simulink model "QuadCopter"  (R2022b)
settings: Solver=ode45  StartTime=0.0  StopTime=500  MaxStep=0.01  RelTol=1e-3
StopFcn:
  | plot3dir(out.X_LQR.x1_or_X__LQR_,out.X_LQR.x2_or_Y, out.X_LQR.x3_or_Z);
  | plot3dir(out.X_MPC.x1_or_X_MPC_,out.X_MPC.x2_or_Y,out.X_MPC.x3_or_Z)
values from neighbouring files (symbols this model uses):
  Fmpc = [0 0 0.003136 0 0 0 0.0020575296 0 0 0 0.0012845056 0 ... (480 elements, 40x12)]    [Fmpc.mat]    (also in FmpcNew.mat = [-6.41677792694e-13 -2.592942847e-12 12.5317858023 -7.722638; dataMPC.m = 2*SuN'*Qbar*Sx)
  g = 9.8    [A.mat]    (also in dataLQR.m)
  Hmpc = [2.0029864 0 0 0 0.00268248 0 0 0 0.00237888 0 0 0 ... (1600 elements, 40x40)]    [Hmpc.mat]    (also in HmpcNew.mat = [2.75081323273 -2.14300187551e-15 -2.22961409187e-14 -3.9742; dataMPC.m = (Hmpc + Hmpc')/2)
  Ix = 0.005    [A.mat]    (also in dataLQR.m)
  Iy = 0.005    [A.mat]    (also in dataLQR.m)
  Iz = 0.009    [A.mat]    (also in dataLQR.m)
  K = [1.7040962205e-15 -3.44587222128e-18 0.005 -1.12753414634e-18 -5.98079995663e-16 -0.005 -2.65215557868e-18 5.41102545065e-19 2 -9.36752747927e-18 -1.48674599099e-17 1.40946704004e-18 ... (48 elements, 4x12)]    [K.mat]
  kf = 1e-05    [A.mat]    (also in dataLQR.m)
  km = 1e-07    [A.mat]    (also in dataLQR.m)
  l = 0.2    [A.mat]    (also in dataLQR.m)
  M = 0.5    [A.mat]    (also in dataLQR.m)
libraries: PID_costum x4
CloseFcn:
  | plot3dir(out.X_LQR.x1_or_X__LQR_,out.X_LQR.x2_or_Y, out.X_LQR.x3_or_Z);
  | plot3dir(out.X_MPC.x1_or_X_MPC_,out.X_MPC.x2_or_Y,out.X_MPC.x3_or_Z)
settings Model: Creator=asoltanieh  LastModifiedBy=asoltanieh

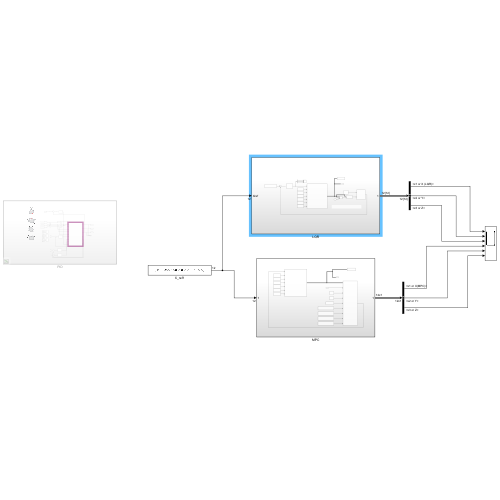
[thumbnail: Simulink's stored preview of the top-level diagram]
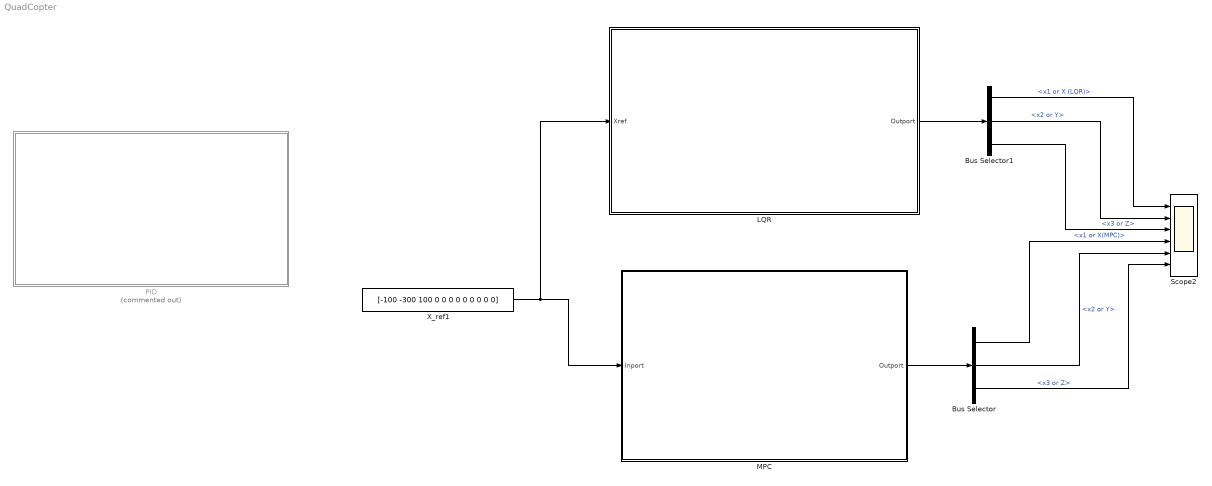
== system QuadCopter ==
  Bus Selector : BusSelector  OutputSignals=x1 or X(MPC),x2 or Y,x3 or Z
  Bus Selector1 : BusSelector  OutputSignals=x1 or X (LQR),x2 or Y,x3 or Z
  LQR : Subsystem
  MPC : Subsystem
  PID : Subsystem  Commented=on
  Scope2 : Scope  NumInputPorts=6
  X_ref1 : Constant  Value=[-100 -300 100 0 0 0 0 0 0 0 0 0]
  wires:
  Bus Selector/2 -> Scope2/5  "<x2 or Y>"
  Bus Selector/1 -> Scope2/4  "<x1 or X(MPC)>"
  Bus Selector/3 -> Scope2/6  "<x3 or Z>"
  MPC/1(Outport) -> Bus Selector/1
  LQR/1(Outport) -> Bus Selector1/1
  Bus Selector1/3 -> Scope2/3  "<x3 or Z>"
  Bus Selector1/1 -> Scope2/1  "<x1 or X (LQR)>"
  Bus Selector1/2 -> Scope2/2  "<x2 or Y>"
  X_ref1/1 -> LQR/1(Xref), MPC/1(Inport)

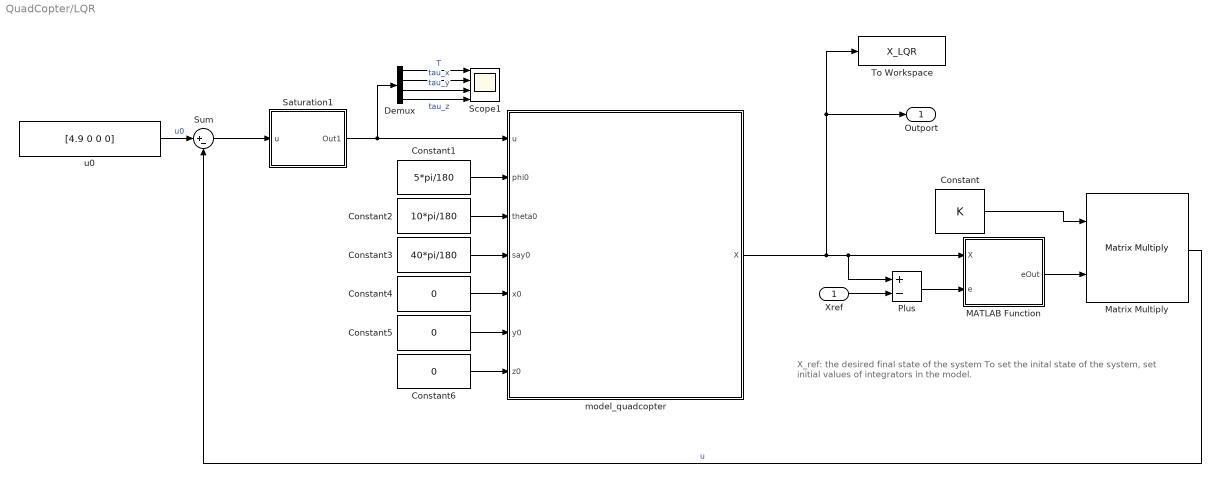
== system QuadCopter/LQR ==
  note: X_ref: the desired final state of the system
      |
      | To set the inital state of the system, set initial values of integrators in the model.
  Xref : Inport
  Constant : Constant  Value=K
  Constant1 : Constant  Value=5*pi/180
  Constant2 : Constant  Value=10*pi/180
  Constant3 : Constant  Value=40*pi/180
  Constant4 : Constant  Value=0
  Constant5 : Constant  Value=0
  Constant6 : Constant  Value=0
  Demux : Demux
  MATLAB Function : MATLAB Function  TreatAsAtomicUnit=on
  Matrix Multiply : Product  Multiplication=Matrix(*)
  Plus : Sum  Inputs=+-
  Saturation1 : Subsystem
  Scope1 : Scope  NumInputPorts=4
  Sum : Sum  Inputs=|+-
  To Workspace : ToWorkspace  VariableName=X_LQR  SaveFormat=Timeseries  SampleTime=-1
  model_quadcopter : Subsystem
  u0 : Constant  Value=[4.9 0 0 0]
  Outport : Outport
  wires:
  model_quadcopter/1(X) -> MATLAB Function/1(X), Plus/1, Outport/1, To Workspace/1
  Constant/1 -> Matrix Multiply/1
  u0/1 -> Sum/1  "u0"
  Sum/1 -> Saturation1/1(u)
  Plus/1 -> MATLAB Function/2(e)
  Xref/1 -> Plus/2
  Demux/1 -> Scope1/1  "T"
  Demux/2 -> Scope1/2  "tau_x"
  Demux/3 -> Scope1/3  "tau_y"
  Demux/4 -> Scope1/4  "tau_z"
  Matrix Multiply/1 -> Sum/2  "u"
  Constant1/1 -> model_quadcopter/2(phi0)
  Constant3/1 -> model_quadcopter/4(say0)
  Constant2/1 -> model_quadcopter/3(theta0)
  Constant4/1 -> model_quadcopter/5(x0)
  Constant5/1 -> model_quadcopter/6(y0)
  Constant6/1 -> model_quadcopter/7(z0)
  Saturation1/1(Out1) -> Demux/1, model_quadcopter/1(u)
  MATLAB Function/1(eOut) -> Matrix Multiply/2

== system QuadCopter/MPC ==
  Inport : Inport
  Constant : Constant  Value=Hmpc
  Constant1 : Constant  Value=Fmpc
  Constant2 : Constant  Value=0.088946471
  Constant3 : Constant  Value=5*pi/180
  Constant4 : Constant  Value=10*pi/180
  Constant5 : Constant  Value=40*pi/180
  Constant6 : Constant  Value=0
  Constant7 : Constant  Value=0
  Constant8 : Constant  Value=0
  MATLAB Function : MATLAB Function  TreatAsAtomicUnit=on
  To Workspace : ToWorkspace  VariableName=X_MPC  SaveFormat=Timeseries  SampleTime=-1
  model_quadcopter : Subsystem
  u0 : Constant  Value=[4.9 0 0 0]
  umax : Constant  Value=[10; 0.01; 0.01; 0.002]
  umin : Constant  Value=[0; -0.01; -0.01; -0.002]
  uscale : Constant  Value=[0.5; 0.003; 0.003; 0.0006]
  Outport : Outport
  wires:
  MATLAB Function/1(U) -> model_quadcopter/1(u)
  Inport/1 -> MATLAB Function/2(Xref)
  Constant/1 -> MATLAB Function/3(Hmpc)
  Constant1/1 -> MATLAB Function/4(Fmpc)
  u0/1 -> MATLAB Function/6(U0)
  Constant2/1 -> MATLAB Function/5(alpha)
  umin/1 -> MATLAB Function/7(Umin)
  umax/1 -> MATLAB Function/8(Umax)
  uscale/1 -> MATLAB Function/9(uScale)
  model_quadcopter/1(X) -> MATLAB Function/1(X), Outport/1, To Workspace/1
  Constant4/1 -> model_quadcopter/3(theta0)
  Constant3/1 -> model_quadcopter/2(phi0)
  Constant8/1 -> model_quadcopter/7(z0)
  Constant7/1 -> model_quadcopter/6(y0)
  Constant5/1 -> model_quadcopter/4(say0)
  Constant6/1 -> model_quadcopter/5(x0)

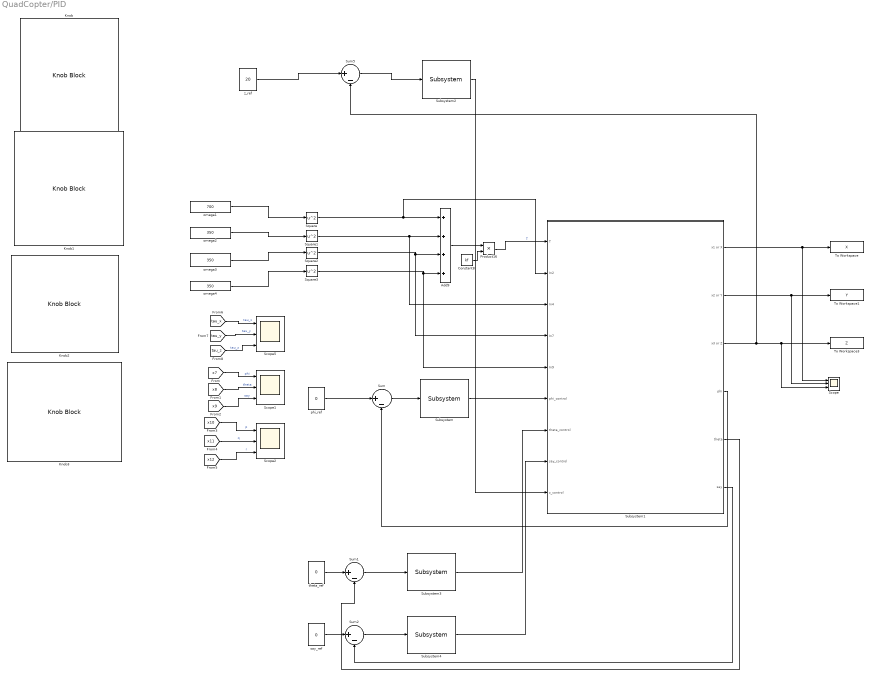
== system QuadCopter/PID ==
  Add9 : Sum  Inputs=++++
  Constant8 : Constant  Value=kf
  Knob{,1..3} (4 alike) : KnobBlock  ScaleMax=700
  Product16 : Product
  Scope{,1..2,5} (4 alike) : Scope  NumInputPorts=3
  Square{,1..3} (4 alike) : Math  Operator=square
  Subsystem : PID_costum/Subsystem  K_P=0.08  K_I=0  K_D=0.032  Sat_value=0.5
  Subsystem1 : Subsystem
  Subsystem2 : PID_costum/Subsystem  K_P=5  K_I=1  K_D=2  Sat_value=10
  Subsystem3 : PID_costum/Subsystem  K_P=0.08  K_I=0  K_D=0.032  Sat_value=0.5
  Subsystem4 : PID_costum/Subsystem  K_P=0.04  K_I=0  K_D=0.07  Sat_value=0.1
  Sum{,1..2,5} (4 alike) : Sum  Inputs=|+-
  To Workspace : ToWorkspace  VariableName=X  SampleTime=-1
  To Workspace1 : ToWorkspace  VariableName=Y  SampleTime=-1
  To Workspace3 : ToWorkspace  VariableName=Z  SampleTime=-1
  omega1 : Constant  Value=700
  omega2 : Constant  Value=350
  omega3 : Constant  Value=350
  omega4 : Constant  Value=350
  phi_ref : Constant  Value=0
  say_ref : Constant  Value=0
  theta_ref : Constant  Value=0
  z_ref : Constant  Value=20
  wires:
  Subsystem1/2(x2 or Y) -> Scope/2, To Workspace1/1
  Product16/1 -> Subsystem1/1(T)  "T"
  [x12] -> Scope2/3  "r"
  [x10] -> Scope2/1  "p"
  Square3/1 -> Subsystem1/5(In9), Add9/4
  [tau_x] -> Scope5/1  "tau_x"
  Subsystem1/4(phi) -> Sum/2
  Subsystem1/3(x3 or Z) -> Sum5/2, Scope/3, To Workspace3/1
  [x11] -> Scope2/2  "q"
  [tau_z] -> Scope5/3  "tau_z"
  [tau_y] -> Scope5/2  "tau_y"
  Square2/1 -> Subsystem1/4(In7), Add9/3
  [x7] -> Scope1/1  "phi"
  Square/1 -> Subsystem1/2(In2), Add9/1
  Subsystem1/6(say) -> Sum2/2
  z_ref/1 -> Sum5/1
  [x9] -> Scope1/3  "say"
  omega1/1 -> Square/1
  Add9/1 -> Product16/1
  Square1/1 -> Subsystem1/3(In4), Add9/2
  Constant8/1 -> Product16/2
  phi_ref/1 -> Sum/1
  say_ref/1 -> Sum2/1
  Subsystem1/1(x1 or X) -> Scope/1, To Workspace/1
  Subsystem/1 -> Subsystem1/6(phi_control)
  Sum/1 -> Subsystem/1
  omega4/1 -> Square3/1
  omega3/1 -> Square2/1
  Sum1/1 -> Subsystem3/1
  Sum5/1 -> Subsystem2/1
  Subsystem3/1 -> Subsystem1/7(theta_control)
  omega2/1 -> Square1/1
  Subsystem1/5(theta) -> Sum1/2
  Subsystem4/1 -> Subsystem1/8(say_control)
  theta_ref/1 -> Sum1/1
  Subsystem2/1 -> Subsystem1/9(z_control)
  [x8] -> Scope1/2  "theta"
  Sum2/1 -> Subsystem4/1

== system QuadCopter/LQR/Saturation1 ==
  u : Inport
  Demux1 : Demux
  Saturation : Saturate  UpperLimit=10  LowerLimit=0
  Saturation1 : Saturate  UpperLimit=0.01  LowerLimit=-0.01
  Saturation2 : Saturate  UpperLimit=0.01  LowerLimit=-0.01
  Saturation3 : Saturate  UpperLimit=0.002  LowerLimit=-0.002
  Vector Concatenate : Concatenate  NumInputs=4
  Out1 : Outport
  wires:
  Vector Concatenate/1 -> Out1/1
  u/1 -> Demux1/1
  Saturation2/1 -> Vector Concatenate/3
  Saturation/1 -> Vector Concatenate/1
  Demux1/1 -> Saturation/1
  Demux1/4 -> Saturation3/1
  Demux1/2 -> Saturation1/1
  Saturation1/1 -> Vector Concatenate/2
  Saturation3/1 -> Vector Concatenate/4
  Demux1/3 -> Saturation2/1

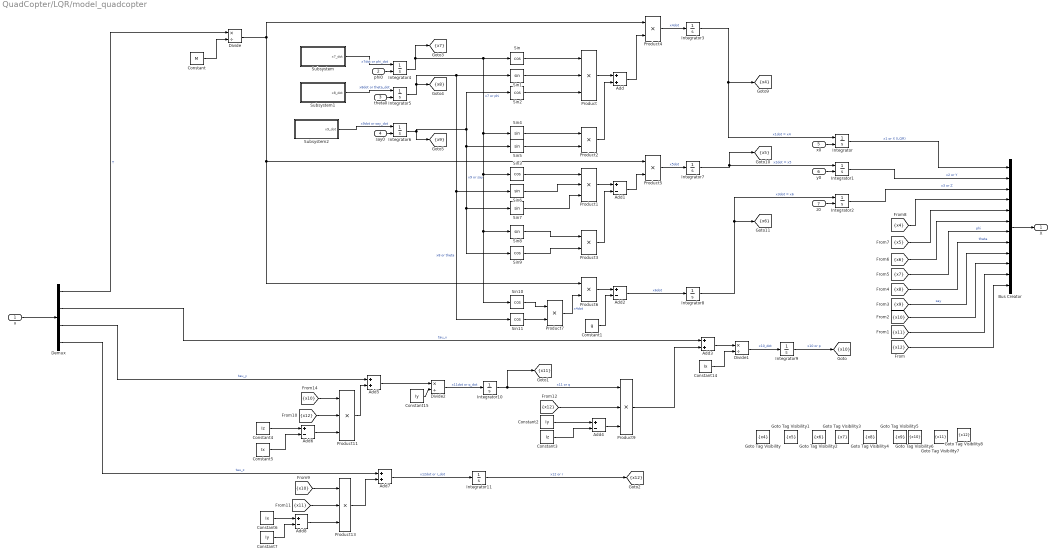
== system QuadCopter/LQR/model_quadcopter ==
  u : Inport
  phi0 : Inport  Port=2
  theta0 : Inport  Port=3
  say0 : Inport  Port=4
  x0 : Inport  Port=5
  y0 : Inport  Port=6
  z0 : Inport  Port=7
  Add{,3,5,7} (4 alike) : Sum
  Add{1..2,4,6,8} (5 alike) : Sum  Inputs=+-
  Bus Creator : BusCreator  Inputs=12
  Constant : Constant  Value=M
  Constant1 : Constant  Value=g
  Constant14 : Constant  Value=Ix
  Constant15 : Constant  Value=Iy
  Constant2 : Constant  Value=Iy
  Constant3 : Constant  Value=Iz
  Constant4 : Constant  Value=Iz
  Constant5 : Constant  Value=Ix
  Constant6 : Constant  Value=Ix
  Constant7 : Constant  Value=Iy
  Demux : Demux
  Divide : Product  Inputs=*/
  Divide1 : Product  Inputs=*/
  Divide2 : Product  Inputs=*/
  Goto Tag Visibility : GotoTagVisibility  GotoTag=x4
  Goto Tag Visibility1 : GotoTagVisibility  GotoTag=x5
  Goto Tag Visibility2 : GotoTagVisibility  GotoTag=x6
  Goto Tag Visibility3 : GotoTagVisibility  GotoTag=x7
  Goto Tag Visibility4 : GotoTagVisibility  GotoTag=x8
  Goto Tag Visibility5 : GotoTagVisibility  GotoTag=x9
  Goto Tag Visibility6 : GotoTagVisibility  GotoTag=x10
  Goto Tag Visibility7 : GotoTagVisibility  GotoTag=x11
  Goto Tag Visibility8 : GotoTagVisibility  GotoTag=x12
  Integrator : Integrator  InitialConditionSource=external  InitialCondition=2
  Integrator1 : Integrator  InitialConditionSource=external  InitialCondition=5
  Integrator{3,7..11} (6 alike) : Integrator
  Integrator2 : Integrator  InitialConditionSource=external  InitialCondition=-1
  Integrator4 : Integrator  InitialConditionSource=external  InitialCondition=20*pi/180
  Integrator5 : Integrator  InitialConditionSource=external  InitialCondition=30*pi/180
  Integrator6 : Integrator  InitialConditionSource=external  InitialCondition=45*pi/180
  Product{,1,9,11,13} (5 alike) : Product  Inputs=3
  Product{2..7} (6 alike) : Product
  Sin{,2..3,9..11} (6 alike) : Trigonometry  Operator=cos
  Sin{1,4..8} (6 alike) : Trigonometry
  Subsystem : Subsystem
  Subsystem1 : Subsystem
  Subsystem2 : Subsystem
  X : Outport
  tag scope: x10=scoped, x11=scoped, x12=scoped, x4=scoped, x5=scoped, x6=scoped, x7=scoped, x8=scoped, x9=scoped
  wires:
  Constant7/1 -> Add8/2
  Product/1 -> Add/1
  Integrator7/1 -> [x5], Integrator1/1  "x2dot = x5"
  Demux/2 -> Add3/1  "tau_x"
  Product7/1 -> Product6/2  "x4dot"
  Add6/1 -> Product11/3
  Add8/1 -> Product13/3
  Demux/4 -> Add7/1  "tau_z"
  Constant14/1 -> Divide1/2
  Divide/1 -> Product6/1, Product5/1, Product4/1
  Integrator6/1 -> Sin2/1, Sin9/1, Sin7/1, Sin5/1, [x9]  "x9 or say"
  Constant3/1 -> Add4/2
  [x10] -> Product13/1
  Divide2/1 -> Integrator10/1  "x11dot or q_dot"
  Add4/1 -> Product9/3
  Subsystem1/1(x8_dot) -> Integrator5/1  "x8dot or theta_dot"
  Product13/1 -> Add7/2
  Constant/1 -> Divide/2
  Integrator10/1 -> [x11], Product9/1  "x11 or q"
  [x11] -> Product13/2
  Sin2/1 -> Product/3
  Constant6/1 -> Add8/1
  Sin/1 -> Product/1
  Sin11/1 -> Product7/2
  Sin6/1 -> Product1/2
  Subsystem/1(x7_dot) -> Integrator4/1  "x7dot or phi_dot"
  Product11/1 -> Add5/2
  Constant2/1 -> Add4/1
  Sin1/1 -> Product/2
  Integrator5/1 -> Sin11/1, Sin6/1, Sin1/1, [x8]  "x8 or theta"
  Sin10/1 -> Product7/1
  Add5/1 -> Divide2/1
  Product3/1 -> Add1/2
  Subsystem2/1(x9_dot) -> Integrator6/1  "x9dot or say_dot"
  Add7/1 -> Integrator11/1  "x12dot or r_dot"
  Add2/1 -> Integrator8/1  "x6dot"
  Add1/1 -> Product5/2
  Constant4/1 -> Add6/1
  Sin3/1 -> Product1/1
  Divide1/1 -> Integrator9/1  "x10_dot"
  [x12] -> Product9/2
  Sin7/1 -> Product1/3
  Product5/1 -> Integrator7/1  "x5dot"
  [x12] -> Product11/2
  Constant15/1 -> Divide2/2
  Product9/1 -> Add3/2
  Integrator4/1 -> Sin10/1, Sin8/1, Sin3/1, Sin4/1, Sin/1, [x7]  "x7 or phi"
  Add3/1 -> Divide1/1
  Integrator3/1 -> [x4], Integrator/1  "x1dot = x4"
  Sin8/1 -> Product3/1
  Sin4/1 -> Product2/1
  Product6/1 -> Add2/1
  [x10] -> Product11/1
  Integrator9/1 -> [x10]  "x10 or p"
  Product1/1 -> Add1/1
  Integrator8/1 -> [x6], Integrator2/1  "x3dot = x6"
  Sin5/1 -> Product2/2
  Constant1/1 -> Add2/2
  Demux/3 -> Add5/1  "tau_y"
  Constant5/1 -> Add6/2
  Add/1 -> Product4/2
  Product2/1 -> Add/2
  Sin9/1 -> Product3/2
  Product4/1 -> Integrator3/1  "x4dot"
  Integrator11/1 -> [x12]  "x12 or r"
  Demux/1 -> Divide/1  "T"
  Bus Creator/1 -> X/1
  u/1 -> Demux/1
  Integrator1/1 -> Bus Creator/2  "x2 or Y"
  Integrator2/1 -> Bus Creator/3  "x3 or Z"
  Integrator/1 -> Bus Creator/1  "x1 or X (LQR)"
  [x4] -> Bus Creator/4
  [x5] -> Bus Creator/5
  [x6] -> Bus Creator/6
  [x7] -> Bus Creator/7  "phi"
  [x8] -> Bus Creator/8  "theta"
  [x9] -> Bus Creator/9  "say"
  [x10] -> Bus Creator/10
  [x11] -> Bus Creator/11
  [x12] -> Bus Creator/12
  phi0/1 -> Integrator4/2
  theta0/1 -> Integrator5/2
  say0/1 -> Integrator6/2
  x0/1 -> Integrator/2
  y0/1 -> Integrator1/2
  z0/1 -> Integrator2/2

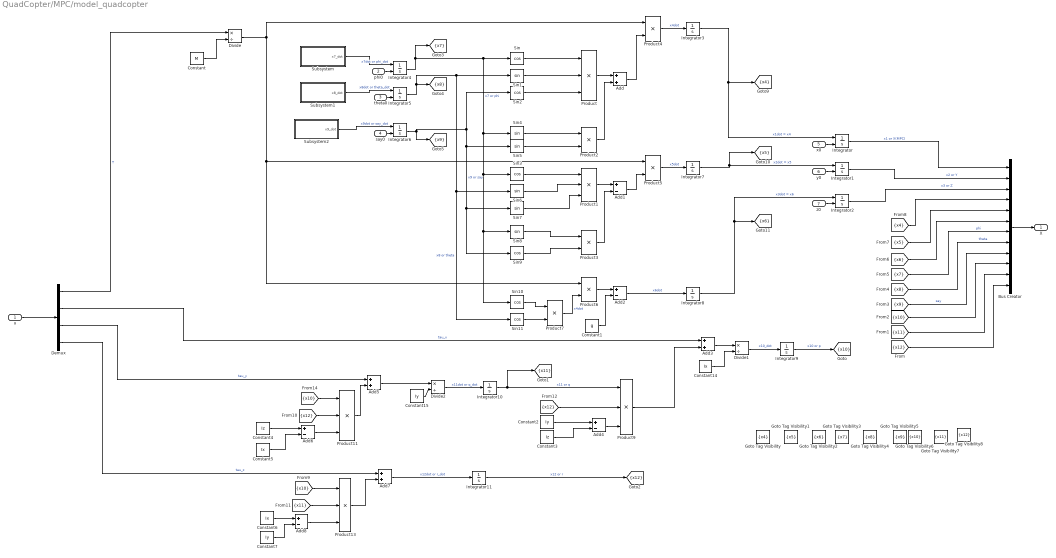
== system QuadCopter/MPC/model_quadcopter ==
  u : Inport
  phi0 : Inport  Port=2
  theta0 : Inport  Port=3
  say0 : Inport  Port=4
  x0 : Inport  Port=5
  y0 : Inport  Port=6
  z0 : Inport  Port=7
  Add{,3,5,7} (4 alike) : Sum
  Add{1..2,4,6,8} (5 alike) : Sum  Inputs=+-
  Bus Creator : BusCreator  Inputs=12
  Constant : Constant  Value=M
  Constant1 : Constant  Value=g
  Constant14 : Constant  Value=Ix
  Constant15 : Constant  Value=Iy
  Constant2 : Constant  Value=Iy
  Constant3 : Constant  Value=Iz
  Constant4 : Constant  Value=Iz
  Constant5 : Constant  Value=Ix
  Constant6 : Constant  Value=Ix
  Constant7 : Constant  Value=Iy
  Demux : Demux
  Divide : Product  Inputs=*/
  Divide1 : Product  Inputs=*/
  Divide2 : Product  Inputs=*/
  Goto Tag Visibility : GotoTagVisibility  GotoTag=x4
  Goto Tag Visibility1 : GotoTagVisibility  GotoTag=x5
  Goto Tag Visibility2 : GotoTagVisibility  GotoTag=x6
  Goto Tag Visibility3 : GotoTagVisibility  GotoTag=x7
  Goto Tag Visibility4 : GotoTagVisibility  GotoTag=x8
  Goto Tag Visibility5 : GotoTagVisibility  GotoTag=x9
  Goto Tag Visibility6 : GotoTagVisibility  GotoTag=x10
  Goto Tag Visibility7 : GotoTagVisibility  GotoTag=x11
  Goto Tag Visibility8 : GotoTagVisibility  GotoTag=x12
  Integrator : Integrator  InitialConditionSource=external  InitialCondition=2
  Integrator1 : Integrator  InitialConditionSource=external  InitialCondition=5
  Integrator{3,7..11} (6 alike) : Integrator
  Integrator2 : Integrator  InitialConditionSource=external  InitialCondition=-1
  Integrator4 : Integrator  InitialConditionSource=external  InitialCondition=20*pi/180
  Integrator5 : Integrator  InitialConditionSource=external  InitialCondition=30*pi/180
  Integrator6 : Integrator  InitialConditionSource=external  InitialCondition=45*pi/180
  Product{,1,9,11,13} (5 alike) : Product  Inputs=3
  Product{2..7} (6 alike) : Product
  Sin{,2..3,9..11} (6 alike) : Trigonometry  Operator=cos
  Sin{1,4..8} (6 alike) : Trigonometry
  Subsystem : Subsystem
  Subsystem1 : Subsystem
  Subsystem2 : Subsystem
  X : Outport
  tag scope: x10=scoped, x11=scoped, x12=scoped, x4=scoped, x5=scoped, x6=scoped, x7=scoped, x8=scoped, x9=scoped
  wires:
  Constant7/1 -> Add8/2
  Product/1 -> Add/1
  Integrator7/1 -> [x5], Integrator1/1  "x2dot = x5"
  Demux/2 -> Add3/1  "tau_x"
  Product7/1 -> Product6/2  "x4dot"
  Add6/1 -> Product11/3
  Add8/1 -> Product13/3
  Demux/4 -> Add7/1  "tau_z"
  Constant14/1 -> Divide1/2
  Divide/1 -> Product6/1, Product5/1, Product4/1
  Integrator6/1 -> Sin2/1, Sin9/1, Sin7/1, Sin5/1, [x9]  "x9 or say"
  Constant3/1 -> Add4/2
  [x10] -> Product13/1
  Divide2/1 -> Integrator10/1  "x11dot or q_dot"
  Add4/1 -> Product9/3
  Subsystem1/1(x8_dot) -> Integrator5/1  "x8dot or theta_dot"
  Product13/1 -> Add7/2
  Constant/1 -> Divide/2
  Integrator10/1 -> [x11], Product9/1  "x11 or q"
  [x11] -> Product13/2
  Sin2/1 -> Product/3
  Constant6/1 -> Add8/1
  Sin/1 -> Product/1
  Sin11/1 -> Product7/2
  Sin6/1 -> Product1/2
  Subsystem/1(x7_dot) -> Integrator4/1  "x7dot or phi_dot"
  Product11/1 -> Add5/2
  Constant2/1 -> Add4/1
  Sin1/1 -> Product/2
  Integrator5/1 -> Sin11/1, Sin6/1, Sin1/1, [x8]  "x8 or theta"
  Sin10/1 -> Product7/1
  Add5/1 -> Divide2/1
  Product3/1 -> Add1/2
  Subsystem2/1(x9_dot) -> Integrator6/1  "x9dot or say_dot"
  Add7/1 -> Integrator11/1  "x12dot or r_dot"
  Add2/1 -> Integrator8/1  "x6dot"
  Add1/1 -> Product5/2
  Constant4/1 -> Add6/1
  Sin3/1 -> Product1/1
  Divide1/1 -> Integrator9/1  "x10_dot"
  [x12] -> Product9/2
  Sin7/1 -> Product1/3
  Product5/1 -> Integrator7/1  "x5dot"
  [x12] -> Product11/2
  Constant15/1 -> Divide2/2
  Product9/1 -> Add3/2
  Integrator4/1 -> Sin10/1, Sin8/1, Sin3/1, Sin4/1, Sin/1, [x7]  "x7 or phi"
  Add3/1 -> Divide1/1
  Integrator3/1 -> [x4], Integrator/1  "x1dot = x4"
  Sin8/1 -> Product3/1
  Sin4/1 -> Product2/1
  Product6/1 -> Add2/1
  [x10] -> Product11/1
  Integrator9/1 -> [x10]  "x10 or p"
  Product1/1 -> Add1/1
  Integrator8/1 -> [x6], Integrator2/1  "x3dot = x6"
  Sin5/1 -> Product2/2
  Constant1/1 -> Add2/2
  Demux/3 -> Add5/1  "tau_y"
  Constant5/1 -> Add6/2
  Add/1 -> Product4/2
  Product2/1 -> Add/2
  Sin9/1 -> Product3/2
  Product4/1 -> Integrator3/1  "x4dot"
  Integrator11/1 -> [x12]  "x12 or r"
  Demux/1 -> Divide/1  "T"
  Bus Creator/1 -> X/1
  u/1 -> Demux/1
  Integrator1/1 -> Bus Creator/2  "x2 or Y"
  Integrator2/1 -> Bus Creator/3  "x3 or Z"
  Integrator/1 -> Bus Creator/1  "x1 or X(MPC)"
  [x4] -> Bus Creator/4
  [x5] -> Bus Creator/5
  [x6] -> Bus Creator/6
  [x7] -> Bus Creator/7  "phi"
  [x8] -> Bus Creator/8  "theta"
  [x9] -> Bus Creator/9  "say"
  [x10] -> Bus Creator/10
  [x11] -> Bus Creator/11
  [x12] -> Bus Creator/12
  phi0/1 -> Integrator4/2
  theta0/1 -> Integrator5/2
  say0/1 -> Integrator6/2
  x0/1 -> Integrator/2
  y0/1 -> Integrator1/2
  z0/1 -> Integrator2/2

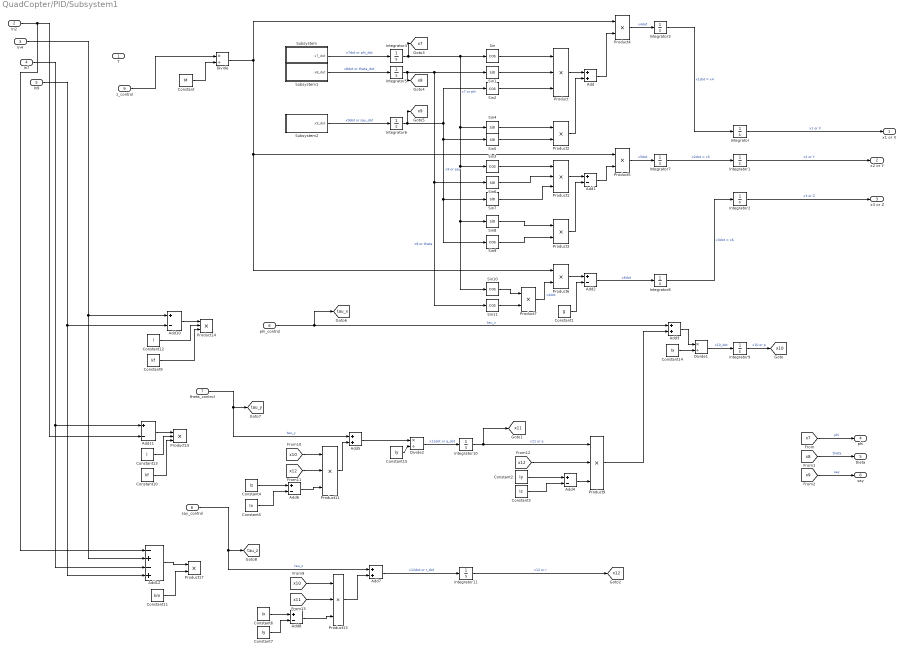
== system QuadCopter/PID/Subsystem1 ==
  T : Inport
  In2 : Inport  Port=2
  In4 : Inport  Port=3
  In7 : Inport  Port=4
  In9 : Inport  Port=5
  phi_control : Inport  Port=6
  theta_control : Inport  Port=7
  say_control : Inport  Port=8
  z_control : Inport  Port=9
  Add{,3,5,7} (4 alike) : Sum
  Add{1..2,4,6,8,10..11} (7 alike) : Sum  Inputs=+-
  Add12 : Sum  Inputs=-+-+
  Constant : Constant  Value=M
  Constant1 : Constant  Value=g
  Constant10 : Constant  Value=kf
  Constant11 : Constant  Value=km
  Constant12 : Constant  Value=l
  Constant13 : Constant  Value=l
  Constant14 : Constant  Value=Ix
  Constant15 : Constant  Value=Iy
  Constant2 : Constant  Value=Iy
  Constant3 : Constant  Value=Iz
  Constant4 : Constant  Value=Iz
  Constant5 : Constant  Value=Ix
  Constant6 : Constant  Value=Ix
  Constant7 : Constant  Value=Iy
  Constant9 : Constant  Value=kf
  Divide : Product  Inputs=*/
  Divide1 : Product  Inputs=*/
  Divide2 : Product  Inputs=*/
  Integrator{,1..3,7..11} (9 alike) : Integrator
  Integrator4 : Integrator  InitialCondition=20*pi/180
  Integrator5 : Integrator  InitialCondition=30*pi/180
  Integrator6 : Integrator  InitialCondition=45*pi/180
  Product{,1,9,11,13..15} (7 alike) : Product  Inputs=3
  Product{2..7,17} (7 alike) : Product
  Sin{,2..3,9..11} (6 alike) : Trigonometry  Operator=cos
  Sin{1,4..8} (6 alike) : Trigonometry
  Subsystem : Subsystem
  Subsystem1 : Subsystem
  Subsystem2 : Subsystem
  x1 or X : Outport
  x2 or Y : Outport  Port=2
  x3 or Z : Outport  Port=3
  phi : Outport  Port=4
  theta : Outport  Port=5
  say : Outport  Port=6
  tag scope: tau_x=global, tau_y=global, tau_z=global, x10=global, x11=global, x12=global, x7=global, x8=global, x9=global
  wires:
  Constant7/1 -> Add8/2
  Product/1 -> Add/1
  Integrator7/1 -> Integrator1/1  "x2dot = x5"
  phi_control/1 -> [tau_x], Add3/1  "tau_x"
  Product7/1 -> Product6/2  "x4dot"
  Add6/1 -> Product11/3
  Add8/1 -> Product13/3
  Add10/1 -> Product14/1
  say_control/1 -> Add7/1, [tau_z]  "tau_z"
  Constant14/1 -> Divide1/2
  Divide/1 -> Product4/1, Product6/1, Product5/1
  Integrator6/1 -> Sin2/1, Sin9/1, Sin7/1, Sin5/1, [x9]  "x9 or say"
  Constant3/1 -> Add4/2
  [x10] -> Product13/1
  Divide2/1 -> Integrator10/1  "x11dot or q_dot"
  Add4/1 -> Product9/3
  Subsystem1/1(x8_dot) -> Integrator5/1  "x8dot or theta_dot"
  Product13/1 -> Add7/2
  Constant9/1 -> Product14/3
  Constant/1 -> Divide/2
  Integrator10/1 -> [x11], Product9/1  "x11 or q"
  Constant12/1 -> Product14/2
  [x11] -> Product13/2
  Sin2/1 -> Product/3
  Constant6/1 -> Add8/1
  Sin/1 -> Product/1
  Sin11/1 -> Product7/2
  Sin6/1 -> Product1/2
  Add11/1 -> Product15/1
  Subsystem/1(x7_dot) -> Integrator4/1  "x7dot or phi_dot"
  Product11/1 -> Add5/2
  Constant2/1 -> Add4/1
  Sin1/1 -> Product/2
  Integrator5/1 -> [x8], Sin11/1, Sin6/1, Sin1/1  "x8 or theta"
  Sin10/1 -> Product7/1
  Add5/1 -> Divide2/1
  In7/1 -> Add12/3, Add11/1
  Constant10/1 -> Product15/3
  Product3/1 -> Add1/2
  Subsystem2/1(x9_dot) -> Integrator6/1  "x9dot or say_dot"
  Add7/1 -> Integrator11/1  "x12dot or r_dot"
  Add2/1 -> Integrator8/1  "x6dot"
  Add1/1 -> Product5/2
  Constant4/1 -> Add6/1
  Integrator1/1 -> x2 or Y/1  "x2 or Y"
  Sin3/1 -> Product1/1
  Divide1/1 -> Integrator9/1  "x10_dot"
  [x12] -> Product9/2
  Sin7/1 -> Product1/3
  Product5/1 -> Integrator7/1  "x5dot"
  [x12] -> Product11/2
  Constant15/1 -> Divide2/2
  Add12/1 -> Product17/1
  Product9/1 -> Add3/2
  Integrator4/1 -> Sin10/1, Sin8/1, Sin3/1, Sin4/1, Sin/1, [x7]  "x7 or phi"
  Constant11/1 -> Product17/2
  Add3/1 -> Divide1/1
  Integrator3/1 -> Integrator/1  "x1dot = x4"
  Sin8/1 -> Product3/1
  Constant13/1 -> Product15/2
  Sin4/1 -> Product2/1
  Product6/1 -> Add2/1
  [x10] -> Product11/1
  Integrator9/1 -> [x10]  "x10 or p"
  In2/1 -> Add12/1, Add11/2
  Product1/1 -> Add1/1
  Integrator8/1 -> Integrator2/1  "x3dot = x6"
  Sin5/1 -> Product2/2
  Constant1/1 -> Add2/2
  theta_control/1 -> Add5/1, [tau_y]  "tau_y"
  Constant5/1 -> Add6/2
  Add/1 -> Product4/2
  Product2/1 -> Add/2
  In4/1 -> Add12/2, Add10/1
  Sin9/1 -> Product3/2
  Product4/1 -> Integrator3/1  "x4dot"
  Integrator11/1 -> [x12]  "x12 or r"
  In9/1 -> Add12/4, Add10/2
  Integrator/1 -> x1 or X/1  "x1 or X"
  Integrator2/1 -> x3 or Z/1  "x3 or Z"
  z_control/1 -> Divide/1
  [x7] -> phi/1  "phi"
  [x8] -> theta/1  "theta"
  [x9] -> say/1  "say"

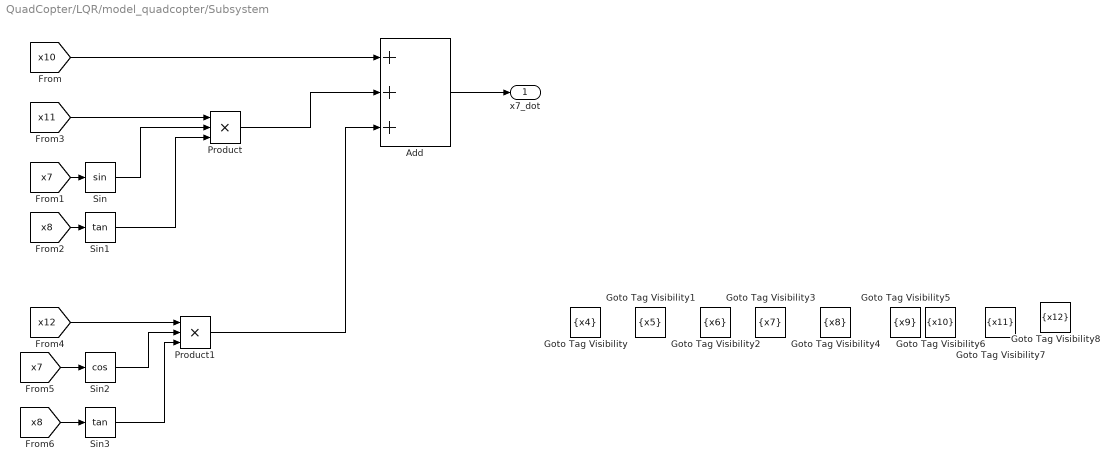
== system QuadCopter/LQR/model_quadcopter/Subsystem ==
  Add : Sum  Inputs=+++
  Goto Tag Visibility : GotoTagVisibility  GotoTag=x4
  Goto Tag Visibility1 : GotoTagVisibility  GotoTag=x5
  Goto Tag Visibility2 : GotoTagVisibility  GotoTag=x6
  Goto Tag Visibility3 : GotoTagVisibility  GotoTag=x7
  Goto Tag Visibility4 : GotoTagVisibility  GotoTag=x8
  Goto Tag Visibility5 : GotoTagVisibility  GotoTag=x9
  Goto Tag Visibility6 : GotoTagVisibility  GotoTag=x10
  Goto Tag Visibility7 : GotoTagVisibility  GotoTag=x11
  Goto Tag Visibility8 : GotoTagVisibility  GotoTag=x12
  Product : Product  Inputs=3
  Product1 : Product  Inputs=3
  Sin : Trigonometry
  Sin1 : Trigonometry  Operator=tan
  Sin2 : Trigonometry  Operator=cos
  Sin3 : Trigonometry  Operator=tan
  x7_dot : Outport
  wires:
  [x10] -> Add/1
  [x11] -> Product/1
  Product/1 -> Add/2
  [x7] -> Sin/1
  Sin/1 -> Product/2
  [x8] -> Sin1/1
  Sin1/1 -> Product/3
  [x12] -> Product1/1
  [x7] -> Sin2/1
  Sin2/1 -> Product1/2
  [x8] -> Sin3/1
  Sin3/1 -> Product1/3
  Product1/1 -> Add/3
  Add/1 -> x7_dot/1

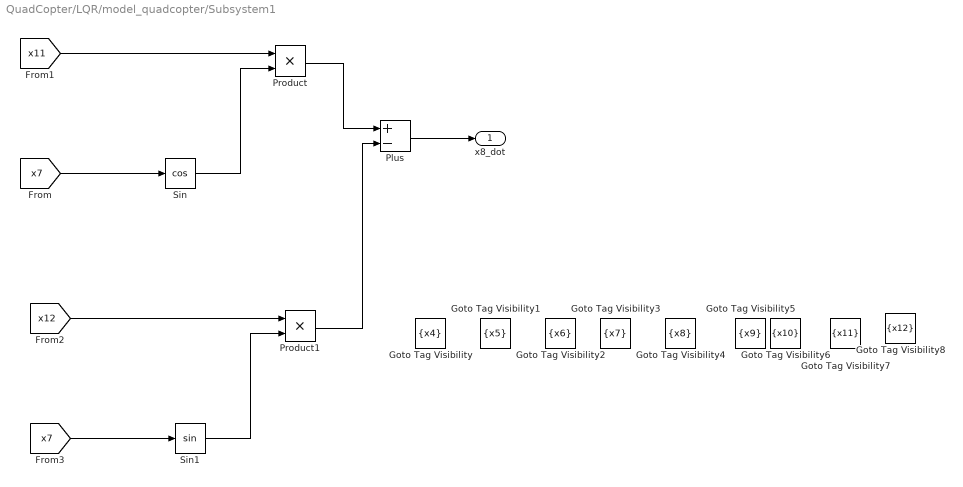
== system QuadCopter/LQR/model_quadcopter/Subsystem1 ==
  Goto Tag Visibility : GotoTagVisibility  GotoTag=x4
  Goto Tag Visibility1 : GotoTagVisibility  GotoTag=x5
  Goto Tag Visibility2 : GotoTagVisibility  GotoTag=x6
  Goto Tag Visibility3 : GotoTagVisibility  GotoTag=x7
  Goto Tag Visibility4 : GotoTagVisibility  GotoTag=x8
  Goto Tag Visibility5 : GotoTagVisibility  GotoTag=x9
  Goto Tag Visibility6 : GotoTagVisibility  GotoTag=x10
  Goto Tag Visibility7 : GotoTagVisibility  GotoTag=x11
  Goto Tag Visibility8 : GotoTagVisibility  GotoTag=x12
  Plus : Sum  Inputs=+-
  Product : Product
  Product1 : Product
  Sin : Trigonometry  Operator=cos
  Sin1 : Trigonometry
  x8_dot : Outport
  wires:
  [x7] -> Sin/1
  Sin/1 -> Product/2
  [x11] -> Product/1
  Product/1 -> Plus/1
  [x12] -> Product1/1
  Sin1/1 -> Product1/2
  [x7] -> Sin1/1
  Product1/1 -> Plus/2
  Plus/1 -> x8_dot/1

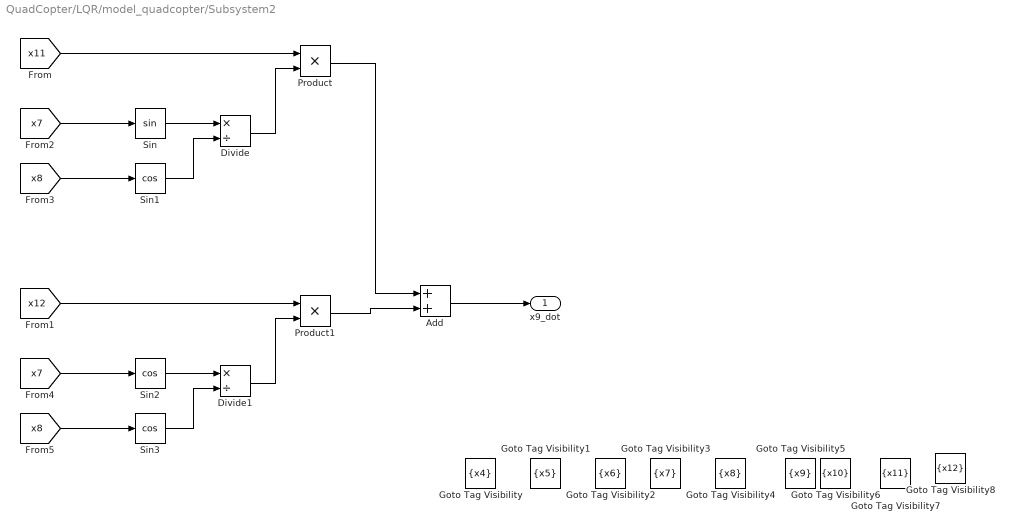
== system QuadCopter/LQR/model_quadcopter/Subsystem2 ==
  Add : Sum
  Divide : Product  Inputs=*/
  Divide1 : Product  Inputs=*/
  Goto Tag Visibility : GotoTagVisibility  GotoTag=x4
  Goto Tag Visibility1 : GotoTagVisibility  GotoTag=x5
  Goto Tag Visibility2 : GotoTagVisibility  GotoTag=x6
  Goto Tag Visibility3 : GotoTagVisibility  GotoTag=x7
  Goto Tag Visibility4 : GotoTagVisibility  GotoTag=x8
  Goto Tag Visibility5 : GotoTagVisibility  GotoTag=x9
  Goto Tag Visibility6 : GotoTagVisibility  GotoTag=x10
  Goto Tag Visibility7 : GotoTagVisibility  GotoTag=x11
  Goto Tag Visibility8 : GotoTagVisibility  GotoTag=x12
  Product : Product
  Product1 : Product
  Sin : Trigonometry
  Sin1 : Trigonometry  Operator=cos
  Sin2 : Trigonometry  Operator=cos
  Sin3 : Trigonometry  Operator=cos
  x9_dot : Outport
  wires:
  [x11] -> Product/1
  [x7] -> Sin/1
  [x8] -> Sin1/1
  Sin/1 -> Divide/1
  Sin1/1 -> Divide/2
  Divide/1 -> Product/2
  Add/1 -> x9_dot/1
  Product/1 -> Add/1
  Product1/1 -> Add/2
  [x12] -> Product1/1
  Divide1/1 -> Product1/2
  Sin3/1 -> Divide1/2
  Sin2/1 -> Divide1/1
  [x8] -> Sin3/1
  [x7] -> Sin2/1

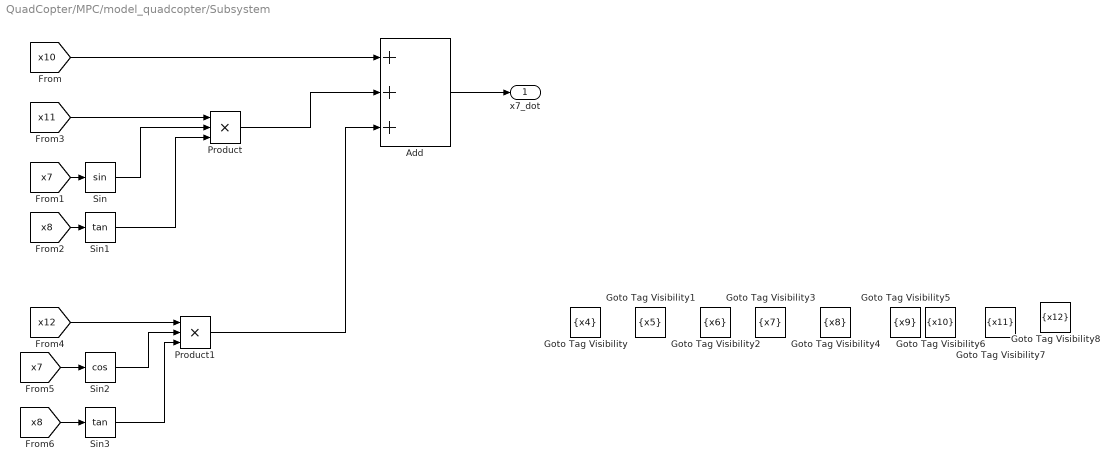
== system QuadCopter/MPC/model_quadcopter/Subsystem ==
  Add : Sum  Inputs=+++
  Goto Tag Visibility : GotoTagVisibility  GotoTag=x4
  Goto Tag Visibility1 : GotoTagVisibility  GotoTag=x5
  Goto Tag Visibility2 : GotoTagVisibility  GotoTag=x6
  Goto Tag Visibility3 : GotoTagVisibility  GotoTag=x7
  Goto Tag Visibility4 : GotoTagVisibility  GotoTag=x8
  Goto Tag Visibility5 : GotoTagVisibility  GotoTag=x9
  Goto Tag Visibility6 : GotoTagVisibility  GotoTag=x10
  Goto Tag Visibility7 : GotoTagVisibility  GotoTag=x11
  Goto Tag Visibility8 : GotoTagVisibility  GotoTag=x12
  Product : Product  Inputs=3
  Product1 : Product  Inputs=3
  Sin : Trigonometry
  Sin1 : Trigonometry  Operator=tan
  Sin2 : Trigonometry  Operator=cos
  Sin3 : Trigonometry  Operator=tan
  x7_dot : Outport
  wires:
  [x10] -> Add/1
  [x11] -> Product/1
  Product/1 -> Add/2
  [x7] -> Sin/1
  Sin/1 -> Product/2
  [x8] -> Sin1/1
  Sin1/1 -> Product/3
  [x12] -> Product1/1
  [x7] -> Sin2/1
  Sin2/1 -> Product1/2
  [x8] -> Sin3/1
  Sin3/1 -> Product1/3
  Product1/1 -> Add/3
  Add/1 -> x7_dot/1

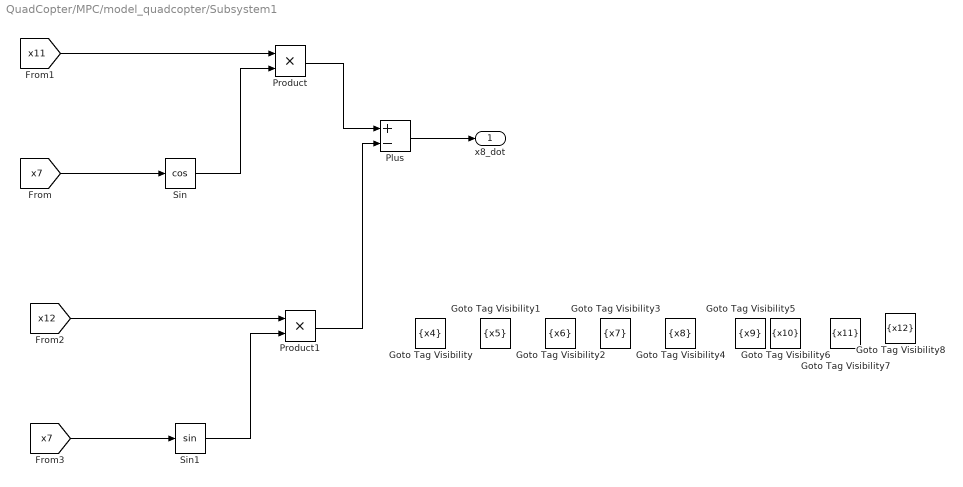
== system QuadCopter/MPC/model_quadcopter/Subsystem1 ==
  Goto Tag Visibility : GotoTagVisibility  GotoTag=x4
  Goto Tag Visibility1 : GotoTagVisibility  GotoTag=x5
  Goto Tag Visibility2 : GotoTagVisibility  GotoTag=x6
  Goto Tag Visibility3 : GotoTagVisibility  GotoTag=x7
  Goto Tag Visibility4 : GotoTagVisibility  GotoTag=x8
  Goto Tag Visibility5 : GotoTagVisibility  GotoTag=x9
  Goto Tag Visibility6 : GotoTagVisibility  GotoTag=x10
  Goto Tag Visibility7 : GotoTagVisibility  GotoTag=x11
  Goto Tag Visibility8 : GotoTagVisibility  GotoTag=x12
  Plus : Sum  Inputs=+-
  Product : Product
  Product1 : Product
  Sin : Trigonometry  Operator=cos
  Sin1 : Trigonometry
  x8_dot : Outport
  wires:
  [x7] -> Sin/1
  Sin/1 -> Product/2
  [x11] -> Product/1
  Product/1 -> Plus/1
  [x12] -> Product1/1
  Sin1/1 -> Product1/2
  [x7] -> Sin1/1
  Product1/1 -> Plus/2
  Plus/1 -> x8_dot/1

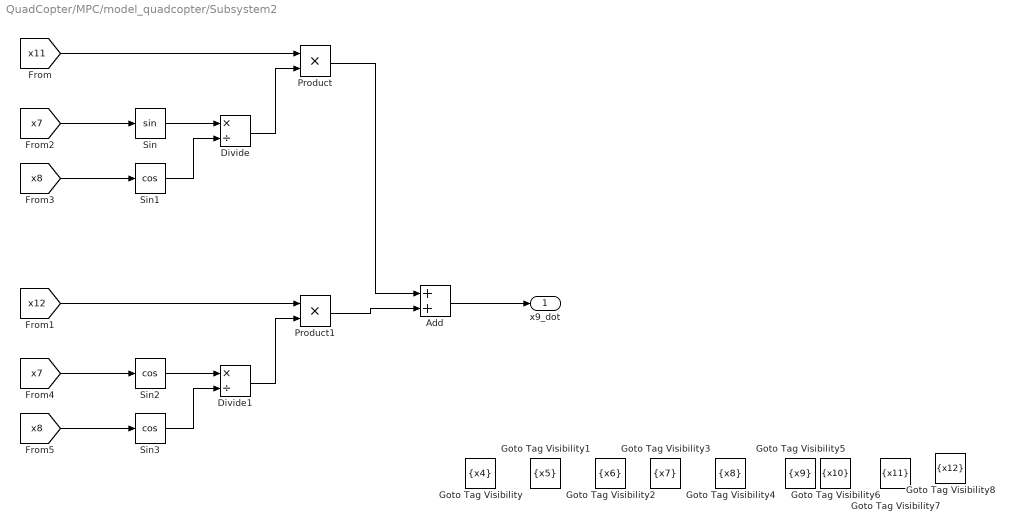
== system QuadCopter/MPC/model_quadcopter/Subsystem2 ==
  Add : Sum
  Divide : Product  Inputs=*/
  Divide1 : Product  Inputs=*/
  Goto Tag Visibility : GotoTagVisibility  GotoTag=x4
  Goto Tag Visibility1 : GotoTagVisibility  GotoTag=x5
  Goto Tag Visibility2 : GotoTagVisibility  GotoTag=x6
  Goto Tag Visibility3 : GotoTagVisibility  GotoTag=x7
  Goto Tag Visibility4 : GotoTagVisibility  GotoTag=x8
  Goto Tag Visibility5 : GotoTagVisibility  GotoTag=x9
  Goto Tag Visibility6 : GotoTagVisibility  GotoTag=x10
  Goto Tag Visibility7 : GotoTagVisibility  GotoTag=x11
  Goto Tag Visibility8 : GotoTagVisibility  GotoTag=x12
  Product : Product
  Product1 : Product
  Sin : Trigonometry
  Sin1 : Trigonometry  Operator=cos
  Sin2 : Trigonometry  Operator=cos
  Sin3 : Trigonometry  Operator=cos
  x9_dot : Outport
  wires:
  [x11] -> Product/1
  [x7] -> Sin/1
  [x8] -> Sin1/1
  Sin/1 -> Divide/1
  Sin1/1 -> Divide/2
  Divide/1 -> Product/2
  Add/1 -> x9_dot/1
  Product/1 -> Add/1
  Product1/1 -> Add/2
  [x12] -> Product1/1
  Divide1/1 -> Product1/2
  Sin3/1 -> Divide1/2
  Sin2/1 -> Divide1/1
  [x8] -> Sin3/1
  [x7] -> Sin2/1

== system QuadCopter/PID/Subsystem1/Subsystem ==
  Add : Sum  Inputs=+++
  Product : Product  Inputs=3
  Product1 : Product  Inputs=3
  Sin : Trigonometry
  Sin1 : Trigonometry  Operator=tan
  Sin2 : Trigonometry  Operator=cos
  Sin3 : Trigonometry  Operator=tan
  x7_dot : Outport
  wires:
  [x10] -> Add/1
  [x11] -> Product/1
  Product/1 -> Add/2
  [x7] -> Sin/1
  Sin/1 -> Product/2
  [x8] -> Sin1/1
  Sin1/1 -> Product/3
  [x12] -> Product1/1
  [x7] -> Sin2/1
  Sin2/1 -> Product1/2
  [x8] -> Sin3/1
  Sin3/1 -> Product1/3
  Product1/1 -> Add/3
  Add/1 -> x7_dot/1

== system QuadCopter/PID/Subsystem1/Subsystem1 ==
  Plus : Sum  Inputs=+-
  Product : Product
  Product1 : Product
  Sin : Trigonometry  Operator=cos
  Sin1 : Trigonometry
  x8_dot : Outport
  wires:
  [x7] -> Sin/1
  Sin/1 -> Product/2
  [x11] -> Product/1
  Product/1 -> Plus/1
  [x12] -> Product1/1
  Sin1/1 -> Product1/2
  [x7] -> Sin1/1
  Product1/1 -> Plus/2
  Plus/1 -> x8_dot/1

== system QuadCopter/PID/Subsystem1/Subsystem2 ==
  Add : Sum
  Divide : Product  Inputs=*/
  Divide1 : Product  Inputs=*/
  Product : Product
  Product1 : Product
  Sin : Trigonometry
  Sin1 : Trigonometry  Operator=cos
  Sin2 : Trigonometry  Operator=cos
  Sin3 : Trigonometry  Operator=cos
  x9_dot : Outport
  wires:
  [x11] -> Product/1
  [x7] -> Sin/1
  [x8] -> Sin1/1
  Sin/1 -> Divide/1
  Sin1/1 -> Divide/2
  Divide/1 -> Product/2
  Add/1 -> x9_dot/1
  Product/1 -> Add/1
  Product1/1 -> Add/2
  [x12] -> Product1/1
  Divide1/1 -> Product1/2
  Sin3/1 -> Divide1/2
  Sin2/1 -> Divide1/1
  [x8] -> Sin3/1
  [x7] -> Sin2/1

== matlab function QuadCopter/LQR/MATLAB Function ==
  data: X input; eOut output; e input
function eOut = shapeError(X, e)
%#codegen
% Shapes the tracking error before it goes to the MPC/LQR:
%   1. wraps the yaw error to [-pi, pi]
%   2. rotates x/y position and velocity errors into the yaw frame
%   3. clips the position error so the controller stays near hover

eMaxXY = 2;    % m, max x/y error shown to the controller
eMaxZ  = 1;    % m, max z error shown to the controller

eOut = e;

% 1. Yaw wrap
eOut(9) = atan2(sin(e(9)), cos(e(9)));

% 2. Rotate into the yaw frame
psi = X(9);
Rz  = [ cos(psi)  sin(psi);
       -sin(psi)  cos(psi)];
eOut(1:2) = Rz*e(1:2);
eOut(4:5) = Rz*e(4:5);

% 3. Clip position error
eOut(1:2) = min(max(eOut(1:2), -eMaxXY), eMaxXY);
eOut(3)   = min(max(eOut(3),   -eMaxZ),  eMaxZ);
end

== matlab function QuadCopter/MPC/MATLAB Function ==
  settings: updateMethod=DISCRETE
  data: X input size=[12 1]; U output; Xref input; Hmpc input; Fmpc input; alpha input; U0 input; Umin input; Umax input; uScale input

function U = myMPC(X, Xref, Hmpc, Fmpc, alpha, ...
                   U0, Umin, Umax, uScale)
%#codegen

N = 15;
nu = 4;
nv = N*nu;

% Previous optimized control sequence
persistent v

if isempty(v)
    v = zeros(nv,1);
end

%% 1. Calculate state tracking error

e = X - Xref;
% Wrap yaw error to [-pi, pi]
e(9) = atan2(sin(e(9)), cos(e(9)));

% Rotate x/y position and velocity errors into the yaw frame
psi = X(9);
Rz  = [ cos(psi)  sin(psi);
       -sin(psi)  cos(psi)];
e(1:2) = Rz*e(1:2);
e(4:5) = Rz*e(4:5);

% Limit position error so the MPC stays near hover
eMaxXY = 2;    % m   (tune: larger = faster but more tilt)
eMaxZ  = 1;    % m
e(1:2) = min(max(e(1:2), -eMaxXY), eMaxXY);
e(3)   = min(max(e(3),   -eMaxZ),  eMaxZ);

%% 2. Normalize actuator constraints

lo = (Umin - U0)./uScale;
hi = (Umax - U0)./uScale;

%% 3. Shift the previous solution

% Move the previous predicted inputs one step forward.
% Keep the last input as the final prediction.

v(1:nv-nu) = v(nu+1:nv);

%% 4. Solve MPC optimization

for iter = 1:150

    % Gradient of quadratic cost
    grad = Hmpc*v + Fmpc*e;

    % Gradient descent
    v = v - alpha*grad;

    % Project inputs onto actuator limits
    for k = 1:N

        idx = (k-1)*nu + (1:nu);

        v(idx) = min(max(v(idx),lo),hi);

    end
end

%% 5. Apply first optimized control input

U = U0 + uScale.*v(1:nu);

end
